simulink model "ModelGridFormingController"  (R2026a)
settings: Solver=ode1be  StopTime=6  FixedStep=gridInverter.vsm.samplingTime  MaxStep=gridInverter.vsm.samplingTime  AbsTol=1e-3
PreLoadFcn:
  | % Parameterize the model
  | TestGridFormingControllerInputParameters;
values from neighbouring files (symbols this model uses):
  localSolverSampleTime = 100e-6    (= 0.0001)    [TestGridFormingControllerInputParameters.m]
undefined symbols (not defined in the file or in its folder): base, Down, gridInverter, Up
libraries: nesl_utility x11, ee_lib x10, fl_lib x4, eeGeneralControl x2, eeSinGeneratorThreePhase x1, ConverterLibrary x1, eePwmGenerator x1
CloseFcn:
  | try, close( 'GridFormingConverterNormalOperation'), end
  | try, close( 'GridFormingConverterActivePowerChange'), end
  | try, close( 'GridFormingConverterReactivePowerChange'), end
  | try, close( 'GridFormingConverterGridVoltageChange'), end
  | try, close( 'GridFormingConverterLocalLoadChange'), end
  | try, close( 'GridFormingConverterSmallGridFreqChange'), end
  | try, close( 'GridFormingConverterLargeGridFreqChange'), end
  | try, close( 'GridFormingConverterFullGridFreqChange'), end
  | try, close( 'GridFormingConverter10DegGridPhaseChange'), end
  | try, close( 'GridFormingConverter60DegGridPhaseChange'), end
  | try, close( 'GridFormingConverterPermanentFault'), end
  | try, close( 'GridFormingConverterTemporaryFault'), end
  | try, close( 'GridFormingConverterActivePowerChangeWithRipple'), end
  | try, close( 'GridFormingConverterIslanding'), end
  | try, close( 'GridFormingConverterDampingEffect'), end
  | try, close( 'GridFormingConverterIntertiaEffect'), end
  | try, close('GridFormingConverterVdControllerBodePlot'), end
  | try, close('GridFormingConverterControllerBodePlot'), end
  | try, close( 'GridFormingConverterThreePhaseFault'), end
  | try, close( 'GridFormingConverterThreePhaseFaultStandard'), end
  | try, close( 'GridFormingConverterCompareFaultRideMethod'), end
  | clear base currentLimitMethodSelected expectedSCR
  | clear grid gridInverter primaryBaseImpedance
  | clear realPowerMethodSelected scrSelected scrFactor
  | clear seconadryBaseImpedance shortCircuit
  | clear simulationTime systemSCR testConditionSelected
  | clear testCondition tout transformer TransmissionLine
  | clear gridVoltageProfileVal gridVoltageProfileTime
  | clear gridFrequencyProfileVal gridFrequencyProfileTime
  | clear gridVoltageProfileVal gridVoltageProfileTime
  | clear gridFrequencyProfileVal gridFrequencyProfileTime
  | clear gridPhaseProfileVal gridPhaseProfileTime
  | clear gfmRealPowerRefProfileVal gfmRealPowerRefProfileTime
  | clear gfmControllerRippleInjectMagVal gfmControllerRippleInjectMagTime
  | clear gfmControllerRippleInjectFreqVal gfmControllerRippleInjectFreqTime
  | clear gfmReactivePowerRefProfileVal gfmReactivePowerRefProfileTime
  | clear localLoadRealProfileVal localLoadRealProfileTime
  | clear localLoadReactiveProfileVal localLoadReactiveProfileTime
  | clear faultTriggerVal faultTriggerTime
  | clear circuitBreakerTripSignalVal circuitBreakerTripSignalTime
  | clear disturbanceTime realPartImpedance  localSolverSampleTime
  | clear SimlogGridFormingConverter temprySampleData
  | clear outValue outputTable plotFlag margintable testOutcome
  | clear realPart  XbyRtempFactor scrFactorXg scrFactorRg scrOut XbyROut systemSCR
  | clear outTable marginTable controllerName dampingArray inertiaConstantArray
  | clear imaginaryPart LogsoutGridFormingConverter faultImpedanceArray
  | clear outData
Description:
  | Design and Analysis of Grid-Forming Converter
settings Model: ExtModeTrigDuration=100  Creator=The MathWorks, Inc.  LastModifiedBy=vsolaise
settings DataIOCC: StateSaveName=tmp_raccel_xout  SignalLoggingName=LogsoutGridFormingConverter  OutputTimes=[0:1.1*3*Voc/(1*2000):1.1*3*Voc/1]  ReturnWorkspaceOutputsName=outData
settings OptimizationCC: EfficientMapNaN2IntZero=off
settings HardwareCC: ProdHWDeviceType=Intel->x86-32 (Windows32)  TargetBitPerPointer=64.0  TargetBitPerSizeT=64.0  TargetBitPerPtrDiffT=64.0  TargetLongLongMode=on  TargetIntDivRoundTo=Zero  TargetEndianess=LittleEndian  TargetWordSize=64.0  TargetHWDeviceType=MATLAB Host  ProdEqTarget=off
settings RTWCC: SystemTargetFile=raccel.tlc  TemplateMakefile=raccel_default_tmf  RTWVerbose=off  RTWUseSimCustomCode=on
settings CodeAppCC: GenerateComments=off  MaxIdLength=128.0  SimulinkBlockComments=off
settings RaccelTargetCC: ExtModeTransport=0.0  ExtModeStaticAllocSize=1000000.0  ENABLE_SLEXEC_SSBRIDGE=1.0  RTWCAPIParams=on  RTWCAPIRootIO=on  MultiwordLength=2048.0
settings SimscapeCC: SimscapeNominalValues="[{\"value\":\"1\",\"unit\":\"A\"},{\"value\":\"1\",\"unit\":\"bar\"},{\"value\":\"1\",\"unit\":\"cm^2\"},{\"value\":\"1\",\"unit\":\"cm^3/s\"},{\"value\":\"1\",\"unit\":\"kJ/kg\"},{\"value\":\"1\",\"unit\":\"kW\"},{\"value\":\"1\",\"unit\":\"l\"},{\"value\":\"1\",\"unit\":\"N\"},{\"value\":\"1\",\"unit\":\"N*m\"},{\"value\":\"1\",\"unit\":\"V\"}]"  SimscapeLogSimulationStatistics=on  SimscapeLogName=SimlogGridFormingConverter  SimscapeLogLimitData=off  SimscapeLogDataHistory=5000.0

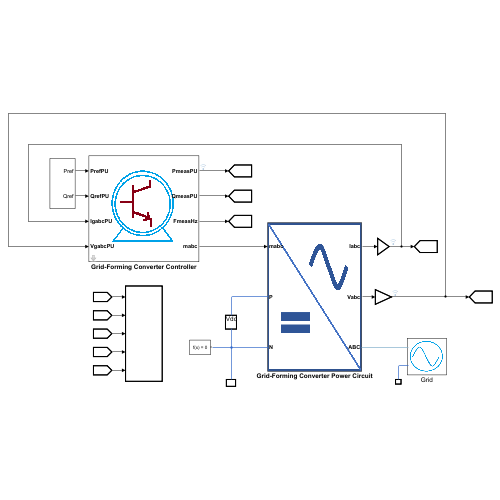
[thumbnail: Simulink's stored preview of the top-level diagram]
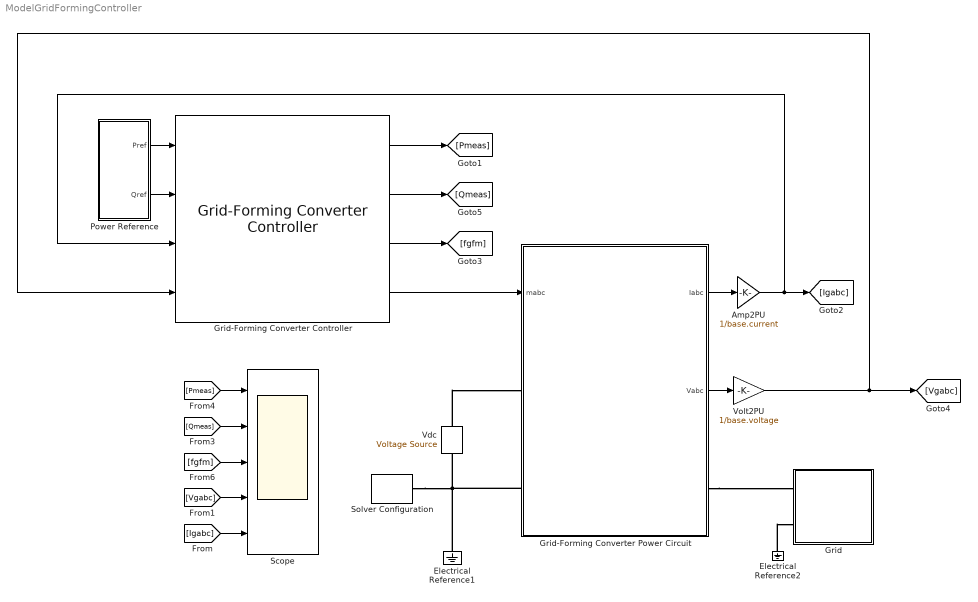
== system ModelGridFormingController ==
  Amp2PU : Gain  Gain=1/base.current
  Electrical Reference1 : fl_lib/Electrical/Electrical Elements/Electrical Reference
  Electrical Reference2 : fl_lib/Electrical/Electrical Elements/Electrical Reference
  Grid : Subsystem
      mask Display: image('$imagefile'); % Use "Edit Image" on toolstrip to change.
  Grid-Forming Converter Controller : ConverterLibrary/Controller/Inverter-Based Resources/Grid-Forming Converter Controller  power=500e3  gridLineVoltage=415  powerFreq=50  dcBusVoltage=1100  measSampleTime=0.0001  powerControl=Virtual Synchronous Machine  activePowerSampleTime=0.0001  droopSlope=0.01  droopT1=0.005  droopT2=0.006  droopTC=0.015  vsmPmeasFilterTC=0.001  vsmFreqDroop=10  vsmInertiaTC=1  vsmDampingConst=1.056  dampingPowerMaxLimit=0.7  dampingPowerMinLimit=-0.6  freqMeasTimeConst=0.15  freqOption=Grid Frequency Measurement  voltreference=1  QVoltFilterTC=0.001  QVoltDroop=0.3  lowVoltageSupportGain=1.5  currentLimit=Virtual Impedance  maxSatCurrentLimit=1.4  maxVICurrentLimit=1.2  ctLimitVirtualImp=2.0625e-1  ctLimitXbyR=13.2  ctLimitDelayTime=0.001  currentSatTime=0.001  currentVITimeConst=0.001  modeTransferTime=10*gridInverter.controller.CurrentControlSampleTime  voltControlTs=0.0001  vdPGain=0.3  VdIGain=180  VdMaxCt=1.8  VdMinCt=-1.8  VqPGain=0.3  VqIGain=180  VqMaxCt=1.8  VqMinCt=-1.8  vdvqLPFTimeConst=0.005  currentControlTs=0.0001  filterInductance=1.0964e-4  IdPGain=1.5  IdIGain=10  IqPGain=1.5  IqIGain=10
      settings: SourceProductName=Simscape Power Converter Components
  Grid-Forming Converter Power Circuit : Subsystem
      mask Display: image('$imagefile'); % Use "Edit Image" on toolstrip to change.
  Power Reference : Subsystem
  Scope : Scope  NumInputPorts=5
      settings: Title=Active Power Measured in pu  ActiveDisplayYMinimum=-0.18492062532329751  ActiveDisplayYMaximum=1.0233144736966111
  Solver Configuration : nesl_utility/Solver Configuration  PhysicalDomain=network_engine_domain  SubClassName=solver  LeftPortType=input  RightPortType=generic  Tones=[]  Harmonics=[]  SimulateNoise=off  Profile=off  UseLocalSampling=off  EnableSwitchedLinearOptims=on  FrequencyDomain=off  UseCCode=off  RelTol=0.001  AbsTol=1e-06  MinStep=1e-09  ToWorkspace=off  RevertToSquareIcSolve=off  NumHomotopyIterations=100  PhasorMode=off  PhasorModeNumHarmonics=1  ConsistencySolver=NEWTON_FTOL  CanonicalOrdering=UNORDERED  OptimizeIntermediates=UNOPTIMIZED  IndexReductionMethod=DerivativeReplacement  DoDC=off  ResidualTolerance=1e-09  ConsistencyTolSource=GLOBAL  ConsistencyAbsTol=0.001  ConsistencyRelTol=0.001  ConsistencyTolFactor=0.001  UseLocalSolver=on  LocalSolverChoice=NE_BACKWARD_EULER_ADVANCER  ResolveIndetEquations=on  FunctionEvalNumThread=1  LocalSolverSampleTime=100e-6  DoFixedCost=on  MaxNonlinIter=3  MaxModeIter=2  ComputeImpulses=off  ImpulseIterations=2  LinearAlgebra=auto  LinearAlgebraNumThread=0  EquationFormulation=NE_TIME_EF  DelaysMemoryBudget=1024  AutomaticFiltering=on  FilteringTimeConstant=0.001  PartitionStorageMethod=AS_NEEDED  PartitionMemoryBudget=1024  PartitionMethod=ROBUST  MultibodyUseLocalSolver=off  MultibodyLocalSolverChoice=ODE1  MultibodyLocalSolverSampleTime=0.001
  Vdc : ee_lib/Sources/Voltage Source  dc_voltage=gridInverter.DCVoltage V  ac_voltage=0 V  ac_shift=0 rad  ac_frequency=0 Hz  noise_mode=ee.enum.sources.noise.Disabled  PSD=0 V^2/Hz  sample_time=1e-3 s  repeatability=ee.enum.sources.repeatability.NotRepeatable  user_seed=0  auto_seed=3499211588  i_specify=off  i_priority=None  i=0 A  i_nominal_specify=off  i_nominal_value=1  i_nominal_unit=A  v_specify=off  v_priority=None  v=0 V  v_nominal_specify=off  v_nominal_value=1  v_nominal_unit=V
  Volt2PU : Gain  Gain=1/base.voltage
  wires:
  [Pmeas] -> Scope/1
  [Qmeas] -> Scope/2
  [fgfm] -> Scope/3
  [Vgabc] -> Scope/4
  [Igabc] -> Scope/5
  Power Reference/1(Pref) -> Grid-Forming Converter Controller/1
  Power Reference/2(Qref) -> Grid-Forming Converter Controller/2
  Grid-Forming Converter Controller/3 -> [fgfm]
  Grid-Forming Converter Power Circuit/1(Iabc) -> Amp2PU/1
  Volt2PU/1 -> Grid-Forming Converter Controller/4, [Vgabc]
  Grid-Forming Converter Power Circuit/2(Vabc) -> Volt2PU/1
  Amp2PU/1 -> Grid-Forming Converter Controller/3, [Igabc]
  Grid-Forming Converter Controller/4 -> Grid-Forming Converter Power Circuit/1(mabc)
  Grid-Forming Converter Controller/2 -> [Qmeas]
  Grid-Forming Converter Controller/1 -> [Pmeas]
  connections:
  Electrical Reference2/LConn1 -- Grid/LConn2
  Vdc/LConn1 -- Grid-Forming Converter Power Circuit/LConn1
  Grid-Forming Converter Power Circuit/LConn2 -- Solver Configuration/RConn1 -- Electrical Reference1/LConn1 -- Vdc/RConn1
  Grid-Forming Converter Power Circuit/RConn1 -- Grid/LConn1

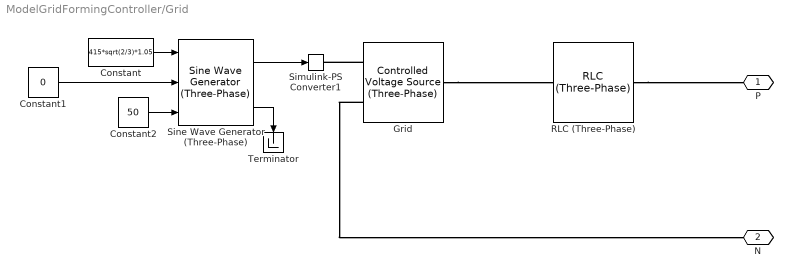
== system ModelGridFormingController/Grid ==
  Constant : Constant  Value=415*sqrt(2/3)*1.05
  Constant1 : Constant  Value=0
  Constant2 : Constant  Value=50
  Grid : ee_lib/Sources/Controlled Voltage Source (Three-Phase)  input_option=ee.enum.inputType.instantaneous  FRated=60 Hz
  RLC (Three-Phase) : ee_lib/Passive/RLC Assemblies/RLC (Three-Phase)  port_option=ee.enum.threePhasePort.composite  component_structure=ee.enum.rlc.structure.R  R=0.1 Ohm  L=1e-3 H  C=1e-6 F  R_parasitic=0 Ohm  G_parasitic=0 1/Ohm  IL_specify=off  IL_priority=High  IL=[0, 0, 0] A  IL_nominal_specify=off  IL_nominal_value=1  IL_nominal_unit=A  VC_specify=off  VC_priority=High  VC=[0, 0, 0] V  VC_nominal_specify=off  VC_nominal_value=1  VC_nominal_unit=V
  Simulink-PS Converter1 : nesl_utility/Simulink-PS Converter  PhysicalDomain=network_engine_domain  SubClassName=ps_input  LeftPortType=input  RightPortType=output  PseudoPeriodic=off  Frequencies=[]  NoiseDistribution=none  NoiseParameters=[]  Unit=1  AffineConversion=off  FilteringAndDerivatives=provide  SimscapeFilterOrder=1  InputFilterTimeConstant=0.001  UdotUserProvided=0
  Sine Wave Generator (Three-Phase) : eeSinGeneratorThreePhase/Sine Wave Generator (Three-Phase)  Ts=100e-6
  Terminator : Terminator
  P : PMIOPort  Side=Left
  N : PMIOPort  Port=2  Side=Left
  wires:
  Sine Wave Generator (Three-Phase)/1 -> Simulink-PS Converter1/1
  Sine Wave Generator (Three-Phase)/2 -> Terminator/1
  Constant2/1 -> Sine Wave Generator (Three-Phase)/3
  Constant1/1 -> Sine Wave Generator (Three-Phase)/2
  Constant/1 -> Sine Wave Generator (Three-Phase)/1
  connections:
  Grid/LConn1 -- Simulink-PS Converter1/RConn1
  Grid/LConn2 -- N/RConn1
  Grid/RConn1 -- RLC (Three-Phase)/LConn1
  RLC (Three-Phase)/RConn1 -- P/RConn1

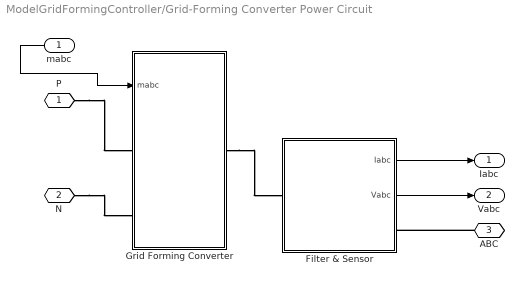
== system ModelGridFormingController/Grid-Forming Converter Power Circuit ==
  mabc : Inport
  Filter & Sensor : Subsystem
      mask Display: image('$imagefile'); % Use "Edit Image" on toolstrip to change.
  Grid Forming Converter : Subsystem  Variant=on  VariantControlMode=label  VariantControl=Grid-Forming Converter Power Circuit  LabelModeActiveChoice=Average
  P : PMIOPort  Side=Left
  N : PMIOPort  Port=2  Side=Left
  ABC : PMIOPort  Port=3  Side=Right
  Iabc : Outport
  Vabc : Outport  Port=2
  wires:
  Filter & Sensor/1(Iabc) -> Iabc/1
  Filter & Sensor/2(Vabc) -> Vabc/1
  mabc/1 -> Grid Forming Converter/1(mabc)
  connections:
  ABC/RConn1 -- Filter & Sensor/RConn1
  P/RConn1 -- Grid Forming Converter/LConn1
  N/RConn1 -- Grid Forming Converter/LConn2
  Grid Forming Converter/RConn1 -- Filter & Sensor/LConn1

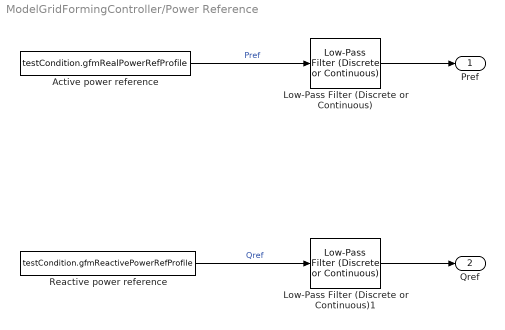
== system ModelGridFormingController/Power Reference ==
  Active power reference : FromWorkspace  VariableName=testCondition.gfmRealPowerRefProfile  SampleTime=localSolverSampleTime  OutputAfterFinalValue=Holding final value
  Low-Pass Filter (Discrete or Continuous) : eeGeneralControl/Low-Pass Filter (Discrete or Continuous)  K=1  T=5e-2  B=inf  A=-inf  init_option=Inherited from block input  x0=0  Ts=-1
  Low-Pass Filter (Discrete or Continuous)1 : eeGeneralControl/Low-Pass Filter (Discrete or Continuous)  K=1  T=5e-2  B=inf  A=-inf  init_option=Inherited from block input  x0=0  Ts=-1
  Reactive power reference : FromWorkspace  VariableName=testCondition.gfmReactivePowerRefProfile  SampleTime=localSolverSampleTime  OutputAfterFinalValue=Holding final value
  Pref : Outport
  Qref : Outport  Port=2
  wires:
  Active power reference/1 -> Low-Pass Filter (Discrete or Continuous)/1  "Pref"
  Reactive power reference/1 -> Low-Pass Filter (Discrete or Continuous)1/1  "Qref"
  Low-Pass Filter (Discrete or Continuous)/1 -> Pref/1
  Low-Pass Filter (Discrete or Continuous)1/1 -> Qref/1

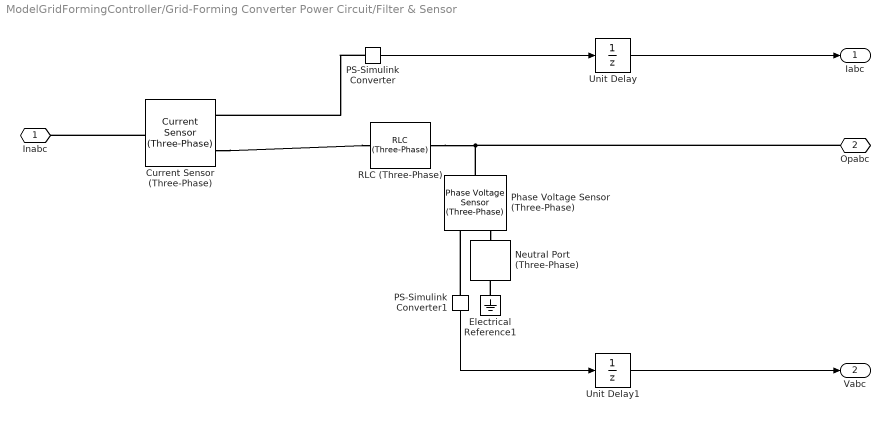
== system ModelGridFormingController/Grid-Forming Converter Power Circuit/Filter & Sensor ==
  Current Sensor (Three-Phase) : ee_lib/Sensors & Transducers/Current Sensor (Three-Phase)  port_option=ee.enum.threePhasePort.composite
  Electrical Reference1 : fl_lib/Electrical/Electrical Elements/Electrical Reference
  Neutral Port (Three-Phase) : ee_lib/Connectors & References/Neutral Port (Three-Phase)  port_option=ee.enum.threePhasePort.composite  G_parasitic=1e-12 1/Ohm
  PS-Simulink Converter : nesl_utility/PS-Simulink Converter  PhysicalDomain=network_engine_domain  SubClassName=ps_output  LeftPortType=input  RightPortType=output  PseudoPeriodic=off  Frequencies=[]  VectorFormat=inherit  Unit=inherit  AffineConversion=off
  PS-Simulink Converter1 : nesl_utility/PS-Simulink Converter  PhysicalDomain=network_engine_domain  SubClassName=ps_output  LeftPortType=input  RightPortType=output  PseudoPeriodic=off  Frequencies=[]  VectorFormat=inherit  Unit=inherit  AffineConversion=off
  Phase Voltage Sensor (Three-Phase) : ee_lib/Sensors & Transducers/Phase Voltage Sensor (Three-Phase)  port_option=ee.enum.threePhasePort.composite
  RLC (Three-Phase) : ee_lib/Passive/RLC Assemblies/RLC (Three-Phase)  port_option=ee.enum.threePhasePort.composite  component_structure=ee.enum.rlc.structure.SeriesRL  R=gridInverter.lineResistance Ohm  L=gridInverter.L H  C=1e-6 F  R_parasitic=0 Ohm  G_parasitic=0 1/Ohm  IL_specify=off  IL_priority=High  IL=[0, 0, 0] A  IL_nominal_specify=off  IL_nominal_value=1  IL_nominal_unit=A  VC_specify=off  VC_priority=High  VC=[0, 0, 0] V  VC_nominal_specify=off  VC_nominal_value=1  VC_nominal_unit=V
  Unit Delay : UnitDelay  SampleTime=-1
  Unit Delay1 : UnitDelay  SampleTime=-1
  Inabc : PMIOPort  Side=Left
  Opabc : PMIOPort  Port=2  Side=Right
  Iabc : Outport
  Vabc : Outport  Port=2
  wires:
  PS-Simulink Converter1/1 -> Unit Delay1/1
  Unit Delay/1 -> Iabc/1
  PS-Simulink Converter/1 -> Unit Delay/1
  Unit Delay1/1 -> Vabc/1
  connections:
  PS-Simulink Converter1/LConn1 -- Phase Voltage Sensor (Three-Phase)/RConn1
  Current Sensor (Three-Phase)/RConn2 -- RLC (Three-Phase)/LConn1
  Current Sensor (Three-Phase)/LConn1 -- Inabc/RConn1
  PS-Simulink Converter/LConn1 -- Current Sensor (Three-Phase)/RConn1
  Phase Voltage Sensor (Three-Phase)/LConn1 -- Opabc/RConn1 -- RLC (Three-Phase)/RConn1
  Phase Voltage Sensor (Three-Phase)/RConn2 -- Neutral Port (Three-Phase)/LConn1
  Electrical Reference1/LConn1 -- Neutral Port (Three-Phase)/RConn1

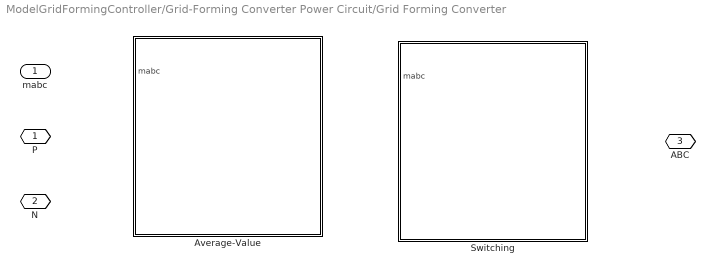
== system ModelGridFormingController/Grid-Forming Converter Power Circuit/Grid Forming Converter ==
  mabc : Inport
  Average-Value : Subsystem  VariantControl=Average
  Switching : Subsystem  VariantControl=Switching
  P : PMIOPort  Side=Left
  N : PMIOPort  Port=2  Side=Left
  ABC : PMIOPort  Port=3  Side=Right

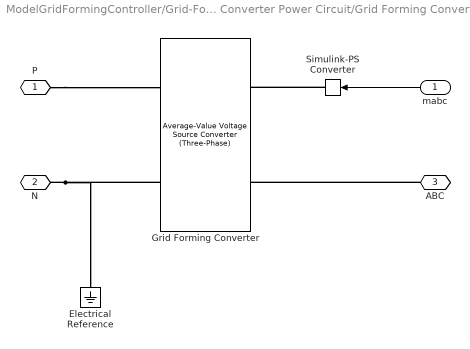
== system ModelGridFormingController/Grid-Forming Converter Power Circuit/Grid Forming Converter/Average-Value ==
  mabc : Inport
  Electrical Reference : fl_lib/Electrical/Electrical Elements/Electrical Reference
  Grid Forming Converter : ee_lib/Semiconductors & Converters/Converters/Average-Value Voltage Source Converter (Three-Phase)  port_option=ee.enum.threePhasePort.composite  enable_block_pulses_input=false  krec=0.01 Ohm  frequency_option=ee.enum.converters.frequency.variable  input_option=ee.enum.converters.inputOption.ModWave  FRated=50 Hz  losses_parameterization=ee.enum.converters.losses.fixed  Pfixed=10 W  ks=0.01  kc1=1.7 V  kc2=0.01 Ohm  Ploss_vect=[100, 800, 1870, 3250, 4900] W  Irms_vect=[10, 100, 200, 300, 400] A  Vdc_nom=300 V  thermal_mass=30000 J/K  temperature_specify=off  temperature_priority=High  temperature=298.15 K  temperature_nominal_specify=off  temperature_nominal_value=1  temperature_nominal_unit=K
  Simulink-PS Converter : nesl_utility/Simulink-PS Converter  PhysicalDomain=network_engine_domain  SubClassName=ps_input  LeftPortType=input  RightPortType=output  PseudoPeriodic=off  Frequencies=[]  NoiseDistribution=none  NoiseParameters=[]  Unit=1  AffineConversion=off  FilteringAndDerivatives=provide  SimscapeFilterOrder=1  InputFilterTimeConstant=0.001  UdotUserProvided=0
  P : PMIOPort  Side=Left
  N : PMIOPort  Port=2  Side=Left
  ABC : PMIOPort  Port=3  Side=Right
  wires:
  mabc/1 -> Simulink-PS Converter/1
  connections:
  N/RConn1 -- Electrical Reference/LConn1 -- Grid Forming Converter/RConn2
  P/RConn1 -- Grid Forming Converter/RConn1
  Simulink-PS Converter/RConn1 -- Grid Forming Converter/LConn1
  ABC/RConn1 -- Grid Forming Converter/LConn2

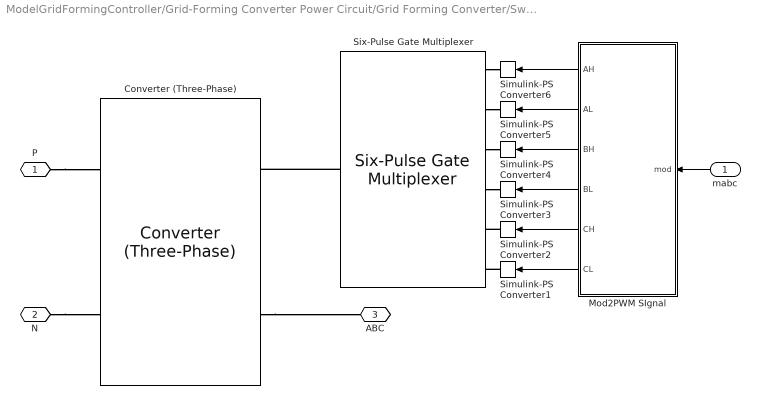
== system ModelGridFormingController/Grid-Forming Converter Power Circuit/Grid Forming Converter/Switching ==
  mabc : Inport
  Converter (Three-Phase) : ee_lib/Semiconductors & Converters/Converters/Converter (Three-Phase)  port_option=ee.enum.threePhasePort.composite  fidelity_option=ee.enum.converters.fidelity.detailed  device_type=ee.enum.converters.switchingdevice.ideal  showThermalPort=false  K=0  Vth=0.5 V  Vgt=1 V  Vgt_off=-1 V  Ih=1 A  Vf=0.8 V  Ron=0.001 Ohm  Rds=0.001 Ohm  Goff=1e-6 1/Ohm  Eon_scalar=22.86e-3 J  Eoff_scalar=17.14e-3 J  Eoff_natural_commutation=10e-3 J  Voff=300 V  Iout_scalar=600 A  onCurrentMeasDelay=0 s  useCurrentFromPreviousCycle=false  useVoltageFromPreviousCycle=false  diode_param=ee.enum.converters.protectiondiode.nodynamics  diode_Vf=0.01 V  diode_Ron=0.0001 Ohm  diode_Goff=1e-5 1/Ohm  diode_C=50 nF  diode_iRM=-235 A  diode_iF=300 A  diode_idot=-50 A/us  diode_trr_param=ee.enum.converters.diodetrr.trr_factor  diode_trr_factor=3  diode_trr=15 us  diode_Qrr=1500 s*uA  diode_rec_loss_model=ee.enum.diode.reverseRecoveryModel.fixed  diode_ErecVal=0 J  diode_scaleWithIandV=false  diode_ErecMat=zeros(2, 3) J  diode_TjrecVec=[298.15, 398.15] K  diode_IfrecVec=[.1, 1, 10] A  diode_IrecVal=10 A  diode_VrecVal=10 V  diode_tFilter=1 / 1000 / 100 s  thermal_network_parameterization=ee.enum.thermalNetworkTopology.external  Rth=[.08, .5] K/W  Rth_Cauer=[.08, .1, .5] K/W  Rth_Foster=[.08, .14, .22, .16] K/W  thermal_mass_parameterization=ee.enum.thermalNetwork.timeconstant  thermal_mass=[.01, .5] J/K  thermal_mass_Cauer=[.01, .1, .5] J/K  thermal_mass_Foster=[.001, .005, .05, .5] J/K  thermal_time_constant=[.001, .2] s  thermal_time_constant_Cauer=[.001, .1, .2] s  thermal_time_constant_Foster=[7e-05, .0007, .01, .08] s  thermal_mass_initial_temperatures=[25, 25] degC  thermal_mass_initial_temperatures_Cauer=[25, 25, 25] degC  junction_thermal_mass=0.01 J/K  Tvec_initial_Foster=[25, 25, 25, 25] degC  snubber_type=ee.enum.converters.snubber.exclude  Cs=1e-7 F  Rs=0.1 Ohm  Vce_loss=[0, 150, 300] V
  Mod2PWM SIgnal : Subsystem
  Simulink-PS Converter{1..6} (6 alike) : nesl_utility/Simulink-PS Converter  PhysicalDomain=network_engine_domain  SubClassName=ps_input  LeftPortType=input  RightPortType=output  PseudoPeriodic=off  Frequencies=[]  NoiseDistribution=none  NoiseParameters=[]  Unit=1  AffineConversion=off  FilteringAndDerivatives=provide  SimscapeFilterOrder=1  InputFilterTimeConstant=0.001  UdotUserProvided=0
  Six-Pulse Gate Multiplexer : ee_lib/Semiconductors & Converters/Converters/Six-Pulse Gate Multiplexer  port_option=ee.enum.controlport.ps
  P : PMIOPort  Side=Left
  N : PMIOPort  Port=2  Side=Left
  ABC : PMIOPort  Port=3  Side=Right
  wires:
  Mod2PWM SIgnal/6(CL) -> Simulink-PS Converter1/1
  Mod2PWM SIgnal/5(CH) -> Simulink-PS Converter2/1
  Mod2PWM SIgnal/4(BL) -> Simulink-PS Converter3/1
  Mod2PWM SIgnal/3(BH) -> Simulink-PS Converter4/1
  Mod2PWM SIgnal/2(AL) -> Simulink-PS Converter5/1
  Mod2PWM SIgnal/1(AH) -> Simulink-PS Converter6/1
  mabc/1 -> Mod2PWM SIgnal/1(mod)
  connections:
  Converter (Three-Phase)/LConn2 -- ABC/RConn1
  Six-Pulse Gate Multiplexer/LConn4 -- Simulink-PS Converter3/RConn1
  Six-Pulse Gate Multiplexer/LConn3 -- Simulink-PS Converter4/RConn1
  N/RConn1 -- Converter (Three-Phase)/RConn2
  Six-Pulse Gate Multiplexer/LConn1 -- Simulink-PS Converter6/RConn1
  Simulink-PS Converter1/RConn1 -- Six-Pulse Gate Multiplexer/LConn6
  Simulink-PS Converter2/RConn1 -- Six-Pulse Gate Multiplexer/LConn5
  Six-Pulse Gate Multiplexer/LConn2 -- Simulink-PS Converter5/RConn1
  P/RConn1 -- Converter (Three-Phase)/RConn1
  Six-Pulse Gate Multiplexer/RConn1 -- Converter (Three-Phase)/LConn1

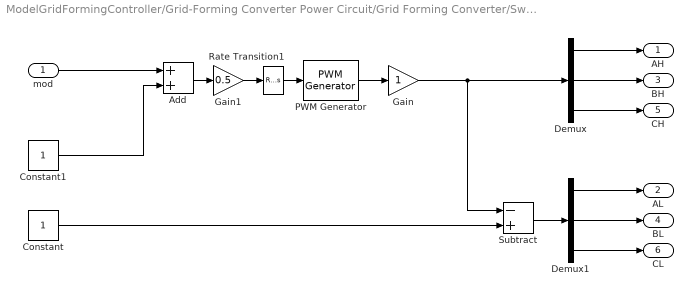
== system ModelGridFormingController/Grid-Forming Converter Power Circuit/Grid Forming Converter/Switching/Mod2PWM SIgnal ==
  mod : Inport
  Add : Sum
  Constant : Constant
  Constant1 : Constant
  Demux : Demux  Outputs=3
  Demux1 : Demux  Outputs=3
  Gain : Gain
  Gain1 : Gain  Gain=0.5
  PWM Generator : eePwmGenerator/PWM Generator  CarrCount=Up-Down  Tper=1/gridInverter.switchingFrequency  Tdelay=0  Ts=1/(10*gridInverter.switchingFrequency)
  Rate Transition1 : RateTransition  OutPortSampleTime=1/(10*gridInverter.switchingFrequency)
  Subtract : Sum  Inputs=-+
  AH : Outport
  AL : Outport  Port=2
  BH : Outport  Port=3
  BL : Outport  Port=4
  CH : Outport  Port=5
  CL : Outport  Port=6
  wires:
  Demux/3 -> CH/1
  Demux/2 -> BH/1
  Demux1/1 -> AL/1
  Demux/1 -> AH/1
  Demux1/3 -> CL/1
  Demux1/2 -> BL/1
  Constant/1 -> Subtract/2
  Subtract/1 -> Demux1/1
  Rate Transition1/1 -> PWM Generator/1
  Add/1 -> Gain1/1
  mod/1 -> Add/1
  PWM Generator/1 -> Gain/1
  Constant1/1 -> Add/2
  Gain1/1 -> Rate Transition1/1
  Gain/1 -> Subtract/1, Demux/1
